simulink model "m07"  (R2025a)
settings: Solver=FixedStepAuto  StartTime=0.0  StopTime=9  FixedStep=dtsim  MaxStep=dtmax  RelTol=1e-4  AbsTol=1e-6  EnableMultiTasking=on
values from neighbouring files (symbols this model uses):
  gnd_xpnts = linspace(-gnd_rng / 2, gnd_rng / 2, num_xpnts)    [m07_params.m]    (also in m07_params_A2.m = linspace(-gnd_rng/2, gnd_rng/2, num_xpnts))
  gnd_ypnts = linspace(-gnd_rng / 2, gnd_rng / 2, num_ypnts)    [m07_params.m]    (also in m07_params_A2.m = linspace(-gnd_rng/2, gnd_rng/2, num_ypnts))
  gnd_zelev = zeros(num_xpnts, num_ypnts)    [m07_params.m]    (also in m07_params_A2.m)
  ic = []    [m07_params.m]    (also in m07_params_A2.m)
  LxFP0 = 0    [m07_params.m]    (also in m07_params_A2.m)
  LyFP0 = mp.wstep    [m07_params.m]    (also in m07_params_A2.m)
  LzFP0 = 0    [m07_params.m]    (also in m07_params_A2.m)
  mp = block.DialogPrm(1).Data    [m07_anim.m]    (also in m07_anim_A2.m; m07_params.m = []; m07_params_A2.m = [])
  RxFP0 = 0    [m07_params.m]    (also in m07_params_A2.m)
  RyFP0 = -0.1    [m07_params.m]    (also in m07_params_A2.m)
  RzFP0 = 0    [m07_params.m]    (also in m07_params_A2.m)
settings Model: Creator=hgeyer  LastModifiedBy=hgeyer
settings SolverCC: AutoScaleAbsTol=off  AlgebraicLoopSolver=TrustRegion
settings DataIOCC: LimitDataPoints=on  SaveFormat=Array  ReturnWorkspaceOutputs=off
settings OptimizationCC: ExpressionDepthLimit=2147483647.0  LifeSpan=inf
settings DebuggingCC: UnderspecifiedInitializationDetection=Classic  MergeDetectMultiDrivingBlocksExec=none  SolverPrmCheckMsg=warning  UnconnectedInputMsg=warning  UnconnectedOutputMsg=warning  UnconnectedLineMsg=warning  StateNameClashWarn=warning  SFUnexpectedBacktrackingDiag=warning  SFNoUnconditionalDefaultTransitionDiag=warning  SFExecutionAtInitializationDiag=none  ArithmeticOperatorsInVariantConditions=warning
settings HardwareCC: ProdBitPerPointer=32.0  ProdBitPerSizeT=32.0  ProdBitPerPtrDiffT=32.0  ProdLargestAtomicFloat=None  ProdIntDivRoundTo=Undefined  ProdEndianess=Unspecified  ProdWordSize=32.0  ProdHWDeviceType=32-bit Generic
settings ModelReferenceCC: PropagateSignalLabelsOutOfModel=off
settings SFSimCC: SimUseLocalCustomCode=off  CustomCodeUndefinedFunction=UseInterfaceOnly
settings RTWCC: RTWUseLocalCustomCode=off  GPUComputeCapability=3.5
settings CodeAppCC: StateflowObjectComments=on
settings GRTTargetCC: TargetLangStandard=C89/C90 (ANSI)
settings ConfigComp: CovMetricSettings=dw  CovSaveCumulativeToWorkspaceVar=on  CovSaveSingleToWorkspaceVar=on  CovExternalEMLEnable=off

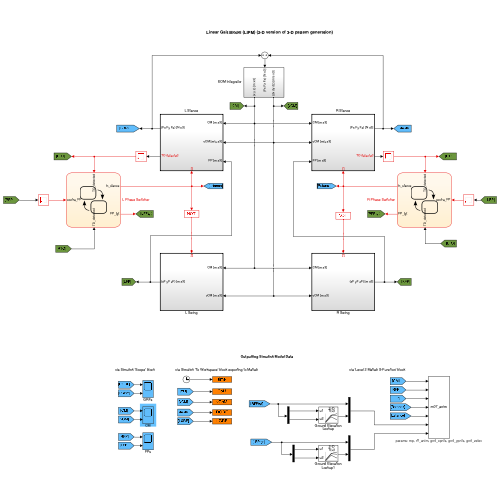
[thumbnail: Simulink's stored preview of the top-level diagram]
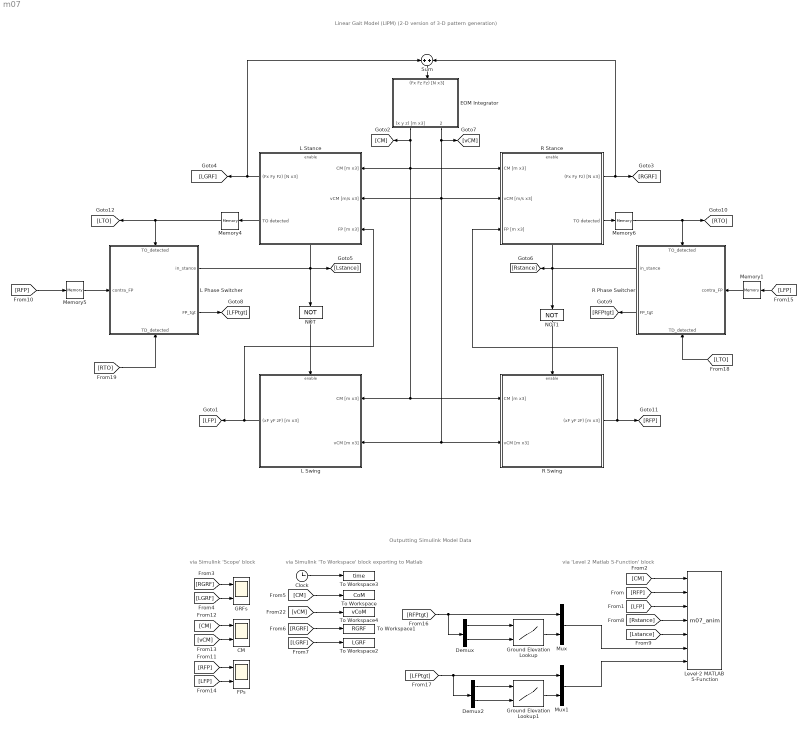
== system m07 ==
  note: via 'Level 2 Matlab S-Function' block
  note: Linear Gait Model (LIPM) (2-D version of 3-D pattern generation)
  note: Outputting Simulink Model Data
  note: via Simulink 'Scope' block
  note: via Simulink 'To Workspace' block exporting to Matlab
  CM : Scope  NumInputPorts=2
      settings: ActiveDisplayYMinimum=-0.72064469784620866  ActiveDisplayYMaximum=5.7194406836575693
  Clock : Clock
  Demux : Demux  Outputs=2
  Demux2 : Demux  Outputs=2
  EOM Integrator : Subsystem
  FPs : Scope  NumInputPorts=2
      settings: ActiveDisplayYMinimum=4.9475948691866245  ActiveDisplayYMaximum=5.0717353469775022  DataLoggingVariableName=ScopeData2
  GRFs : Scope  NumInputPorts=2
      settings: ActiveDisplayYMinimum=-540.42192  ActiveDisplayYMaximum=1399.83708
  Ground Elevation Lookup : Lookup_n-D  BreakpointsForDimension1=gnd_xpnts  BreakpointsForDimension2=gnd_ypnts  Table=gnd_zelev  RemoveProtectionInput=on  InternalRulePriority=Speed  RndMeth=Simplest
      settings: InputPortMap=u0,u1
  Ground Elevation Lookup1 : Lookup_n-D  BreakpointsForDimension1=gnd_xpnts  BreakpointsForDimension2=gnd_ypnts  Table=gnd_zelev  RemoveProtectionInput=on  InternalRulePriority=Speed  RndMeth=Simplest
      settings: InputPortMap=u0,u1
  L Phase Switcher : Stateflow chart  TreatAsAtomicUnit=on
      settings: PortSchema="{\"entries\":[{\"content\":{\"sides\":[{\"content\":{\"connectorIds\":[\"In3\"]},\"type\":\"ConnectorPlacement.EquallySpacedRectSide\",\"uuid\":\"753cae2f-2613-4fde-9c78-e885807ee3e0\"},{\"content\":{\"connectorIds\":[\"Out1\",\"Out2\"],\"side\":\"RIGHT\"},\"type\":\"ConnectorPlacement.EquallySpacedRectSide\",\"uuid\":\"817c0fd6-521f-4f26-adeb-7830d8ec11b0\"},{\"content\":{\"connectorIds\":[\"In1\"],\"side\":\"TOP\"},\"type\":\"ConnectorPlacement.EquallySpacedRectSide\",\"uuid\":\"7f7ae789-722d-4082-ba34-d5db96ef6f27\"},{\"content\":{\"connectorIds\":[\"In2\"],\"side\":\"BOTTOM\"},\"type\":\"ConnectorPlacement.EquallySpacedRectSide\",\"uuid\":\"1a245394-e328-4754-8dab-c57a82d6dff9\"}]},\"type\":\"ConnectorPlacement.EquallySpacedConnector\",\"uuid\":\"c201788b-7347-443d-9526-e208ab85c0f7\"}],\"packageUris\":[\"http://schema.mathworks.com/mf0/Connector/R2020b\"],\"version\":\"1.0\"}"
  L Stance : Subsystem
  L Swing : Subsystem
  Level-2 MATLAB S-Function : M-S-Function  FunctionName=m07_anim  Parameters=mp, rtf_anim, gnd_xpnts, gnd_ypnts, gnd_zelev
      settings: AttributesFormatString=params: %<Parameters>
  Memory{1,4..6} (4 alike) : Memory
  Mux : Mux  Inputs=2
  Mux1 : Mux  Inputs=2
  NOT : Logic  Operator=NOT  AllPortsSameDT=off  OutDataTypeStr=boolean
  NOT1 : Logic  Operator=NOT  AllPortsSameDT=off  OutDataTypeStr=boolean
  R Phase Switcher : Stateflow chart  TreatAsAtomicUnit=on
      settings: PortSchema="{\"entries\":[{\"content\":{\"sides\":[{\"content\":{\"connectorIds\":[\"In3\"]},\"type\":\"ConnectorPlacement.EquallySpacedRectSide\",\"uuid\":\"753cae2f-2613-4fde-9c78-e885807ee3e0\"},{\"content\":{\"connectorIds\":[\"Out1\",\"Out2\"],\"side\":\"RIGHT\"},\"type\":\"ConnectorPlacement.EquallySpacedRectSide\",\"uuid\":\"817c0fd6-521f-4f26-adeb-7830d8ec11b0\"},{\"content\":{\"connectorIds\":[\"In1\"],\"side\":\"TOP\"},\"type\":\"ConnectorPlacement.EquallySpacedRectSide\",\"uuid\":\"7f7ae789-722d-4082-ba34-d5db96ef6f27\"},{\"content\":{\"connectorIds\":[\"In2\"],\"side\":\"BOTTOM\"},\"type\":\"ConnectorPlacement.EquallySpacedRectSide\",\"uuid\":\"1a245394-e328-4754-8dab-c57a82d6dff9\"}]},\"type\":\"ConnectorPlacement.EquallySpacedConnector\",\"uuid\":\"c201788b-7347-443d-9526-e208ab85c0f7\"}],\"packageUris\":[\"http://schema.mathworks.com/mf0/Connector/R2020b\"],\"version\":\"1.0\"}"
  R Stance : Subsystem
  R Swing : Subsystem
  Sum : Sum
  To Workspace : ToWorkspace  VariableName=CoM  SampleTime=0.01
  To Workspace1 : ToWorkspace  VariableName=RGRF  SampleTime=0.01
  To Workspace2 : ToWorkspace  VariableName=LGRF  SampleTime=0.01
  To Workspace3 : ToWorkspace  VariableName=time  SampleTime=0.01
  To Workspace4 : ToWorkspace  VariableName=vCoM  SampleTime=0.01
  wires:
  Sum/1 -> EOM Integrator/1((Fx Fz Fz) [N x3])
  L Stance/1((Fx Fy Fz) [N x3]) -> [LGRF], Sum/1
  R Stance/1((Fx Fy Fz) [N x3]) -> [RGRF], Sum/2
  EOM Integrator/2((dx dy dz) [m/s x3]) -> [vCM], R Swing/2(vCM [m x3]), L Swing/2(vCM [m x3]), R Stance/2(vCM [m/s x3]), L Stance/2(vCM [m/s x3])
  [RFP] -> Level-2 MATLAB S-Function/2
  [LFP] -> Level-2 MATLAB S-Function/3
  [CM] -> Level-2 MATLAB S-Function/1
  [RGRF] -> GRFs/1
  [LGRF] -> GRFs/2
  [CM] -> To Workspace/1
  [RGRF] -> To Workspace1/1
  [LGRF] -> To Workspace2/1
  Clock/1 -> To Workspace3/1
  [Rstance] -> Level-2 MATLAB S-Function/4
  [Lstance] -> Level-2 MATLAB S-Function/5
  L Phase Switcher/1(in_stance) -> NOT/1, [Lstance], L Stance/Enable
  NOT/1 -> L Swing/Enable
  NOT1/1 -> R Swing/Enable
  R Phase Switcher/1(in_stance) -> NOT1/1, R Stance/Enable, [Rstance]
  EOM Integrator/1((x y z) [m x3]) -> [CM], R Swing/1(CM [m x3]), L Swing/1(CM [m x3]), R Stance/1(CM [m x3]), L Stance/1(CM [m x3])
  R Swing/1((xF yF zF) [m x3]) -> R Stance/3(FP [m x3]), [RFP]
  L Swing/1((xF yF zF) [m x3]) -> L Stance/3(FP [m x3]), [LFP]
  [vCM] -> To Workspace4/1
  [CM] -> CM/1
  [vCM] -> CM/2
  [RFP] -> Memory5/1
  [LFP] -> Memory1/1
  Memory1/1 -> R Phase Switcher/3(contra_FP)
  Mux/1 -> Level-2 MATLAB S-Function/6
  Mux1/1 -> Level-2 MATLAB S-Function/7
  R Stance/2(TO detected) -> Memory6/1
  L Stance/2(TO detected) -> Memory4/1
  Memory4/1 -> [LTO], L Phase Switcher/1(TO_detected)
  Memory6/1 -> R Phase Switcher/1(TO_detected), [RTO]
  [LTO] -> R Phase Switcher/2(TD_detected)
  [RTO] -> L Phase Switcher/2(TD_detected)
  Memory5/1 -> L Phase Switcher/3(contra_FP)
  [LFP] -> FPs/2
  [RFP] -> FPs/1
  L Phase Switcher/2(FP_tgt) -> [LFPtgt]
  R Phase Switcher/2(FP_tgt) -> [RFPtgt]
  [RFPtgt] -> Demux/1, Mux/1
  Demux/1 -> Ground Elevation Lookup/1
  Demux/2 -> Ground Elevation Lookup/2
  Ground Elevation Lookup/1 -> Mux/2
  Ground Elevation Lookup1/1 -> Mux1/2
  [LFPtgt] -> Demux2/1, Mux1/1
  Demux2/1 -> Ground Elevation Lookup1/1
  Demux2/2 -> Ground Elevation Lookup1/2

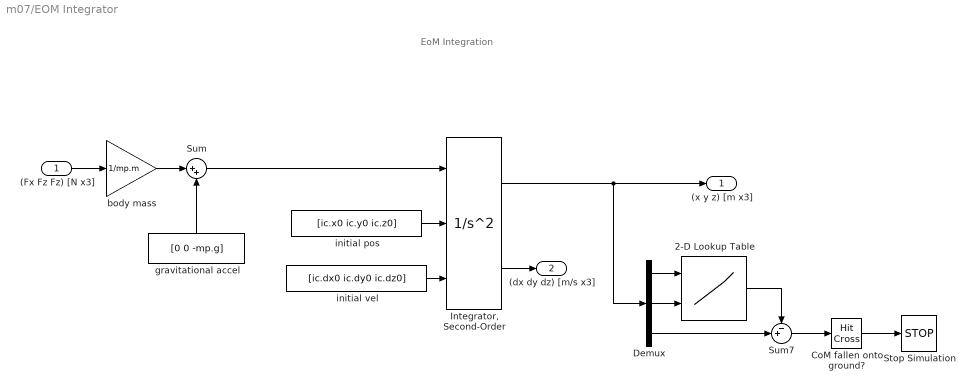
== system m07/EOM Integrator ==
  note: EoM Integration
  (Fx Fz Fz) [N x3] : Inport
  2-D Lookup Table : Lookup_n-D  BreakpointsForDimension1=gnd_xpnts  BreakpointsForDimension2=gnd_ypnts  Table=gnd_zelev  RemoveProtectionInput=on  InternalRulePriority=Speed  RndMeth=Simplest
      settings: InputPortMap=u0,u1
  CoM fallen onto ground? : HitCross  HitCrossingDirection=falling
      settings: AttributesFormatString=offset: %<HitCrossingOffset>
  Demux : Demux  Outputs=3
  "Integrator, Second-Order" : SecondOrderIntegrator  ICSourceX=external  ICSourceDXDT=external
  Stop Simulation : Stop
  Sum : Sum  Inputs=|++
  Sum7 : Sum  Inputs=-+|
  body mass : Gain  Gain=1/mp.m
  gravitational accel : Constant  Value=[0 0 -mp.g]
  initial pos : Constant  Value=[ic.x0 ic.y0 ic.z0]
  initial vel : Constant  Value=[ic.dx0 ic.dy0 ic.dz0]
  (x y z) [m x3] : Outport
  (dx dy dz) [m/s x3] : Outport  Port=2
  wires:
  "Integrator, Second-Order"/1 -> Demux/1, (x y z) [m x3]/1
  initial vel/1 -> "Integrator, Second-Order"/3
  gravitational accel/1 -> Sum/2
  (Fx Fz Fz) [N x3]/1 -> body mass/1
  initial pos/1 -> "Integrator, Second-Order"/2
  "Integrator, Second-Order"/2 -> (dx dy dz) [m/s x3]/1
  Sum/1 -> "Integrator, Second-Order"/1
  body mass/1 -> Sum/1
  CoM fallen onto ground?/1 -> Stop Simulation/1
  Sum7/1 -> CoM fallen onto ground?/1
  Demux/1 -> 2-D Lookup Table/1
  Demux/2 -> 2-D Lookup Table/2
  2-D Lookup Table/1 -> Sum7/1
  Demux/3 -> Sum7/2

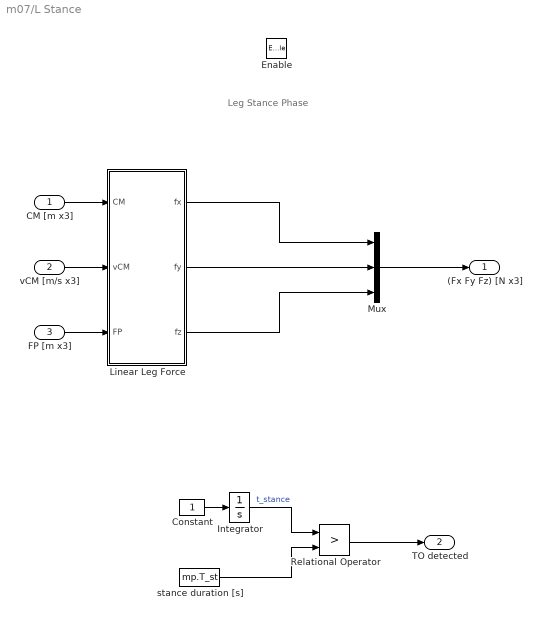
== system m07/L Stance ==
  note: Leg Stance Phase
  CM [m x3] : Inport
  vCM [m/s x3] : Inport  Port=2
  FP [m x3] : Inport  Port=3
  Enable : EnablePort  StatesWhenEnabling=reset
      settings: AttributesFormatString=when enabled: %<StatesWhenEnabling>
  Constant : Constant
  Integrator : Integrator
  Linear Leg Force : MATLAB Function  TreatAsAtomicUnit=on
  Mux : Mux  Inputs=3
  Relational Operator : RelationalOperator  Operator=>  OutDataTypeStr=boolean  RndMeth=Simplest  InputSameDT=off
  stance duration [s] : Constant  Value=mp.T_st
  (Fx Fy Fz) [N x3] : Outport  OutputWhenDisabled=reset  InitialOutput=[0 0 0]
      settings: AttributesFormatString=|
      | when disabled: %<OutputWhenDisabled>
      | initial: %<InitialOutput>
  TO detected : Outport  Port=2  OutputWhenDisabled=reset  InitialOutput=0
      settings: AttributesFormatString=|
      | when disabled: %<OutputWhenDisabled>
      | initial: %<InitialOutput>
  wires:
  Mux/1 -> (Fx Fy Fz) [N x3]/1
  CM [m x3]/1 -> Linear Leg Force/1(CM)
  vCM [m/s x3]/1 -> Linear Leg Force/2(vCM)
  FP [m x3]/1 -> Linear Leg Force/3(FP)
  Linear Leg Force/1(fx) -> Mux/1
  Relational Operator/1 -> TO detected/1
  stance duration [s]/1 -> Relational Operator/2
  Integrator/1 -> Relational Operator/1  "t_stance"
  Constant/1 -> Integrator/1
  Linear Leg Force/2(fy) -> Mux/2
  Linear Leg Force/3(fz) -> Mux/3

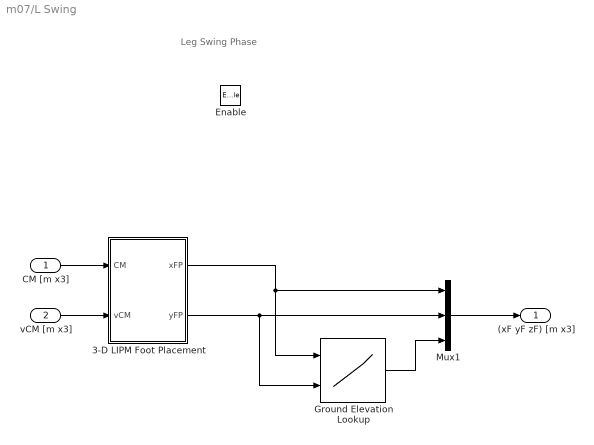
== system m07/L Swing ==
  note: Leg Swing Phase
  CM [m x3] : Inport
  vCM [m x3] : Inport  Port=2
  Enable : EnablePort  StatesWhenEnabling=reset
      settings: AttributesFormatString=when enabled: %<StatesWhenEnabling>
  3-D LIPM Foot Placement : MATLAB Function  TreatAsAtomicUnit=on
  Ground Elevation Lookup : Lookup_n-D  BreakpointsForDimension1=gnd_xpnts  BreakpointsForDimension2=gnd_ypnts  Table=gnd_zelev  RemoveProtectionInput=on  InternalRulePriority=Speed  RndMeth=Simplest
      settings: InputPortMap=u0,u1
  Mux1 : Mux  Inputs=3
  (xF yF zF) [m x3] : Outport  InitialOutput=[LxFP0, LyFP0, LzFP0]
      settings: AttributesFormatString=|
      | initial: %<InitialOutput>
      | when disabled: %<OutputWhenDisabled>
  wires:
  CM [m x3]/1 -> 3-D LIPM Foot Placement/1(CM)
  vCM [m x3]/1 -> 3-D LIPM Foot Placement/2(vCM)
  Ground Elevation Lookup/1 -> Mux1/3
  3-D LIPM Foot Placement/1(xFP) -> Ground Elevation Lookup/1, Mux1/1
  3-D LIPM Foot Placement/2(yFP) -> Ground Elevation Lookup/2, Mux1/2
  Mux1/1 -> (xF yF zF) [m x3]/1

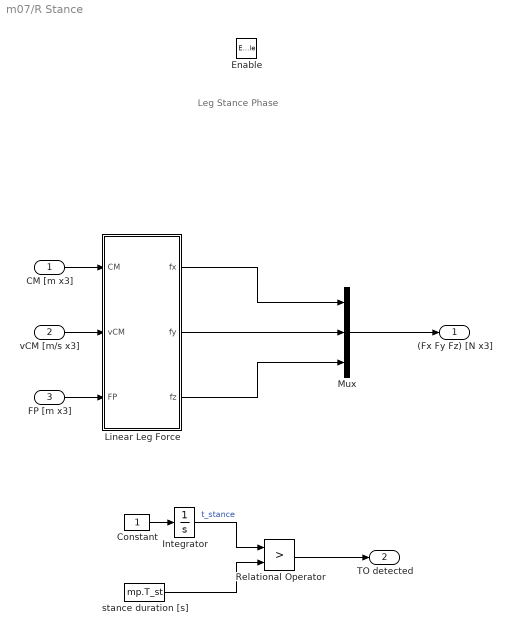
== system m07/R Stance ==
  note: Leg Stance Phase
  CM [m x3] : Inport
  vCM [m/s x3] : Inport  Port=2
  FP [m x3] : Inport  Port=3
  Enable : EnablePort  StatesWhenEnabling=reset
      settings: AttributesFormatString=when enabled: %<StatesWhenEnabling>
  Constant : Constant
  Integrator : Integrator
  Linear Leg Force : MATLAB Function  TreatAsAtomicUnit=on
  Mux : Mux  Inputs=3
  Relational Operator : RelationalOperator  Operator=>  OutDataTypeStr=boolean  RndMeth=Simplest  InputSameDT=off
  stance duration [s] : Constant  Value=mp.T_st
  (Fx Fy Fz) [N x3] : Outport  OutputWhenDisabled=reset  InitialOutput=[0 0 0]
      settings: AttributesFormatString=|
      | when disabled: %<OutputWhenDisabled>
      | initial: %<InitialOutput>
  TO detected : Outport  Port=2  OutputWhenDisabled=reset  InitialOutput=0
      settings: AttributesFormatString=|
      | when disabled: %<OutputWhenDisabled>
      | initial: %<InitialOutput>
  wires:
  Linear Leg Force/1(fx) -> Mux/1
  Mux/1 -> (Fx Fy Fz) [N x3]/1
  CM [m x3]/1 -> Linear Leg Force/1(CM)
  vCM [m/s x3]/1 -> Linear Leg Force/2(vCM)
  FP [m x3]/1 -> Linear Leg Force/3(FP)
  Constant/1 -> Integrator/1
  Integrator/1 -> Relational Operator/1  "t_stance"
  Relational Operator/1 -> TO detected/1
  stance duration [s]/1 -> Relational Operator/2
  Linear Leg Force/2(fy) -> Mux/2
  Linear Leg Force/3(fz) -> Mux/3

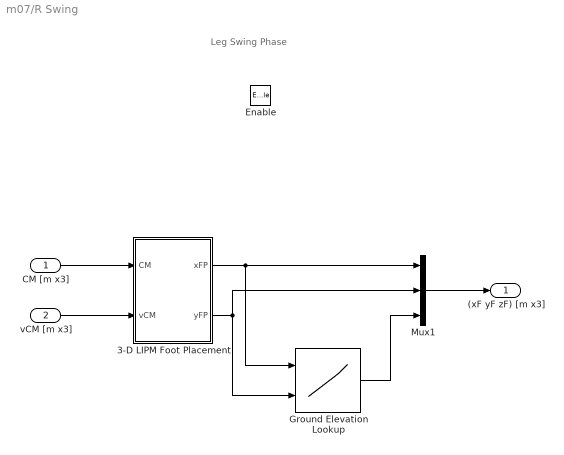
== system m07/R Swing ==
  note: Leg Swing Phase
  CM [m x3] : Inport
  vCM [m x3] : Inport  Port=2
  Enable : EnablePort  StatesWhenEnabling=reset
      settings: AttributesFormatString=when enabled: %<StatesWhenEnabling>
  3-D LIPM Foot Placement : MATLAB Function  TreatAsAtomicUnit=on
  Ground Elevation Lookup : Lookup_n-D  BreakpointsForDimension1=gnd_xpnts  BreakpointsForDimension2=gnd_ypnts  Table=gnd_zelev  RemoveProtectionInput=on  InternalRulePriority=Speed  RndMeth=Simplest
      settings: InputPortMap=u0,u1
  Mux1 : Mux  Inputs=3
  (xF yF zF) [m x3] : Outport  InitialOutput=[RxFP0, RyFP0, RzFP0]
      settings: AttributesFormatString=|
      | initial: %<InitialOutput>
      | when disabled: %<OutputWhenDisabled>
  wires:
  Mux1/1 -> (xF yF zF) [m x3]/1
  CM [m x3]/1 -> 3-D LIPM Foot Placement/1(CM)
  vCM [m x3]/1 -> 3-D LIPM Foot Placement/2(vCM)
  Ground Elevation Lookup/1 -> Mux1/3
  3-D LIPM Foot Placement/1(xFP) -> Ground Elevation Lookup/1, Mux1/1
  3-D LIPM Foot Placement/2(yFP) -> Ground Elevation Lookup/2, Mux1/2

== matlab function m07/R Swing/3-D LIPM Foot Placement ==
  data: CM input; xFP output; vCM input; mp parameter; yFP output
function [xFP, yFP] = fcn(CM, vCM, mp)
%
% FRight Leg Foot Placement in 3-D Linear Inverted Pendulum
%
% hgeyer, Sep 2025
%

% LIPM math terms
w = sqrt(mp.g / mp.z0);
C = cosh(w * mp.T_st);
S = sinh(w * mp.T_st);
D = mp.a * (C-1)^2 + mp.b * (w * S)^2;

% goal state after completing stance at time mp.T_st
x_des = mp.lstep / 2;
dx_des = mp.vtgt;
y_des = mp.wstep / 2;
dy_des = y_des * w * (C - 1) / S;

% initial position and velocity
x0 = -x_des;
dx0 = vCM(1);
y0 = y_des;
dy0 = vCM(2);

% optimal foot placement given cost terms mp.a and mp.b
px = - mp.a * (C - 1) / D * (x_des - C * x0 - S / w * dx0) ...
  - mp.b * w * S / D * (dx_des - S * w * x0 - C * dx0);

py = - mp.a * (C - 1) / D * (y_des - C * y0 - S / w * dy0) ...
  - mp.b * w * S / D * (dy_des - S * w * y0 - C * dy0);

% resulting foot point location in world frame
xFP = CM(1) + mp.lstep / 2 + px;
yFP = CM(2) - mp.wstep / 2 + py;

== matlab function m07/L Swing/3-D LIPM Foot Placement ==
  data: CM input; xFP output; vCM input; mp parameter; yFP output
function [xFP, yFP] = fcn(CM, vCM, mp)
%
% Left Foot Placement in 3-D Linear Inverted Pendulum
%
% hgeyer, Sep 2025
%

% LIPM math terms
w = sqrt(mp.g / mp.z0);
C = cosh(w * mp.T_st);
S = sinh(w * mp.T_st);
D = mp.a * (C-1)^2 + mp.b * (w * S)^2;

% goal state after completing stance at time mp.T_st
x_des = mp.lstep / 2;
dx_des = mp.vtgt;       
y_des = -mp.wstep / 2;   
dy_des = y_des * w * (C - 1) / S;

% initial position and velocity
x0 = -x_des;
dx0 = vCM(1);
y0 = y_des;
dy0 = vCM(2);

% optimal foot placement given cost terms mp.a and mp.b
px = - mp.a * (C - 1) / D * (x_des - C * x0 - S / w * dx0) ...
  - mp.b * w * S / D * (dx_des - S * w * x0 - C * dx0);

py = - mp.a * (C - 1) / D * (y_des - C * y0 - S / w * dy0) ...
  - mp.b * w * S / D * (dy_des - S * w * y0 - C * dy0);

% resulting foot point location in world frame
xFP = CM(1) + mp.lstep / 2 + px;
yFP = CM(2) + mp.wstep / 2 + py;

== matlab function m07/L Stance/Linear Leg Force ==
  data: CM input; fx output; fy output; vCM input; FP input; fz output; mp parameter
function [fx, fy, fz] = fcn(CM, vCM, FP, mp)

% 3-D Linear Gait Leg Force
%
% H. Geyer, Aug 2025

% relative CoM coordinates
xrel = CM(1) - FP(1);
yrel = CM(2) - FP(2);
zrel = CM(3) - FP(3);

% CoM velocity components
dz = vCM(3);

% Leg Force
fz = mp.m * mp.g +  mp.K * (mp.z0 - zrel) - mp.B * dz;
if fz < 0.0   % observe push constraint
    fz = 0.0;
end

fx = xrel / zrel * fz; 
fy = yrel / zrel * fz;

== matlab function m07/R Stance/Linear Leg Force ==
  data: CM input; fx output; fy output; vCM input; FP input; fz output; mp parameter
function [fx, fy, fz] = fcn(CM, vCM, FP, mp)

% 3-D Linear Gait Leg Force
%
% H. Geyer, Aug 2025

% relative CoM coordinates
xrel = CM(1) - FP(1);
yrel = CM(2) - FP(2);
zrel = CM(3) - FP(3);

% CoM velocity components
dz = vCM(3);

% Leg Force
fz = mp.m * mp.g +  mp.K * (mp.z0 - zrel) - mp.B * dz;
if fz < 0.0   % observe push constraint
    fz = 0.0;
end

fx = xrel / zrel * fz; 
fy = yrel / zrel * fz;

== stateflow chart m07/R Phase Switcher ==
  state Stance
    entry:
    in_stance = true;
  state Swing
    entry:
    in_stance = false;
    FP_tgt = contra_FP(1:2) + [mp.lstep; - mp.wstep];
  (default) -> Stance
  Swing -> Stance : [TD_detected]
  Stance -> Swing : [TO_detected]
  data: TO_detected input; TD_detected input; in_stance output; mp parameter; contra_FP input; FP_tgt output

== stateflow chart m07/L Phase Switcher ==
  state Stance
    entry:
    in_stance = true;
  state Swing
    entry:
    in_stance = false;
    FP_tgt = contra_FP(1:2) + [mp.lstep; mp.wstep];
  (default) -> Swing
  Swing -> Stance : [TD_detected]
  Stance -> Swing : [TO_detected]
  data: TO_detected input; TD_detected input; in_stance output; mp parameter; contra_FP input; FP_tgt output
